simulink model "harmosc_det"  (Simulink 4.00)
settings: Solver=ode45  StartTime=0.0  StopTime=100.0  RelTol=1e-3
values from neighbouring files (symbols this model uses):
  c = 0.1    [damposc.m]
  k = k+1    (= 1)    [avarstudy.m]    (also in plotkalout.m = 2)
  m = length(v1)    [collate.m]    (also in damposc.m = 1; kalgen.m = input('Enter number of measurements (or dimension of measure; state9.m = 3; state9_01.mat = 1)
libraries: simulink3 x1
settings Model: BlockReductionOpt=off

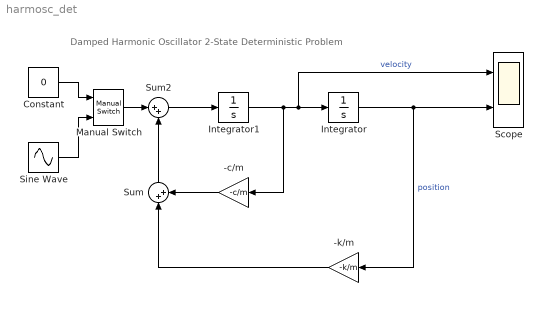
== system harmosc_det ==
  note: Damped Harmonic Oscillator
      | 2-State Deterministic Problem
  -c/m : Gain  Orientation=left  Gain=-c/m  Multiplication=Element-wise(K.*u)  SaturateOnIntegerOverflow=on
  -k/m : Gain  Orientation=left  Gain=-k/m  Multiplication=Element-wise(K.*u)  SaturateOnIntegerOverflow=on
  Constant : Constant  Value=0
  Integrator : Integrator  ExternalReset=none  InitialConditionSource=internal  InitialCondition=10  LimitOutput=off  UpperSaturationLimit=inf  LowerSaturationLimit=-inf  ShowSaturationPort=off  ShowStatePort=off  AbsoluteTolerance=auto
  Integrator1 : Integrator  ExternalReset=none  InitialConditionSource=internal  InitialCondition=0  LimitOutput=off  UpperSaturationLimit=inf  LowerSaturationLimit=-inf  ShowSaturationPort=off  ShowStatePort=off  AbsoluteTolerance=auto
  Manual Switch : simulink3/Nonlinear/Manual Switch  sw=1  action=0
  Scope : Scope  NumInputPorts=2
      settings: TimeRange=auto  YMin=-5~-5  YMax=5~5  SaveToWorkspace=off  SaveName=ScopeData  LimitDataPoints=on  MaxDataPoints=5000
  Sine Wave : Sin  Amplitude=1  Frequency=1  Phase=0  SampleTime=0
  Sum : Sum  Orientation=up  Inputs=|++  SaturateOnIntegerOverflow=on
  Sum2 : Sum  Inputs=|++  SaturateOnIntegerOverflow=on
  wires:
  Integrator1/1 -> -c/m/1, Integrator/1, Scope/1  "velocity"
  -c/m/1 -> Sum/2
  -k/m/1 -> Sum/1
  Integrator/1 -> -k/m/1, Scope/2  "position"
  Sum/1 -> Sum2/2
  Manual Switch/1 -> Sum2/1
  Sum2/1 -> Integrator1/1
  Constant/1 -> Manual Switch/1
  Sine Wave/1 -> Manual Switch/2
